simulink model "model"  (R2015a)
settings: Solver=ode3  StartTime=0.0  StopTime=30.0  RelTol=1e-3
undefined symbols (not defined in the file): MIO, National_Instruments, PCI
libraries: sldrtlib x3
settings Model: SimulationMode=external  ExtModeTrigDuration=1501  Creator=Alunos  LastModifiedBy=Alunos
settings HardwareCC: ProdIntDivRoundTo=Zero  ProdEndianess=LittleEndian  ProdHWDeviceType=Intel->x86/Pentium  TargetIntDivRoundTo=Zero  TargetEndianess=LittleEndian  TargetHWDeviceType=Intel->x86/Pentium
settings RTWCC: SystemTargetFile=rtwin.tlc  TemplateMakefile=rtwin.tmf  Description=Simulink Desktop Real-Time  RTWCompilerOptimization=on
settings CodeAppCC: MaxIdLength=95
settings RTWinTargetCC: TargetPreCompLibLocation=C:\Program Files\MATLAB\R2015a\toolbox\sldrt\lib\win32

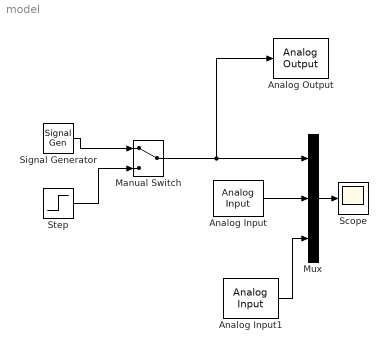
== system model ==
  Analog Input : sldrtlib/Analog Input  SampleTime=0.02  MaxMissedTicks=10  ShowMissedTicks=off  YieldWhenWaiting=off  DrvName=National_Instruments/PCI-MIO-16E-4  DrvAddress=4294967295  DrvOptions=[0 0 0 0 0 0]  Channels=1  RangeMode=1  VoltRange=1  DataType=1
      settings: AttributesFormatString=National Instruments\nPCI-MIO-16E-4 [auto]
  Analog Input1 : sldrtlib/Analog Input  SampleTime=0.02  MaxMissedTicks=10  ShowMissedTicks=off  YieldWhenWaiting=off  DrvName=National_Instruments/PCI-MIO-16E-4  DrvAddress=4294967295  DrvOptions=[0 0 0 0 0 0]  Channels=2  RangeMode=1  VoltRange=1  DataType=1
      settings: AttributesFormatString=National Instruments\nPCI-MIO-16E-4 [auto]
  Analog Output : sldrtlib/Analog Output  SampleTime=0.02  MaxMissedTicks=10  ShowMissedTicks=off  YieldWhenWaiting=off  DrvName=National_Instruments/PCI-MIO-16E-4  DrvAddress=4294967295  DrvOptions=[0 0 0 0 0 0]  Channels=1  RangeMode=1  VoltRange=1  InitialValue=0  FinalValue=0
      settings: AttributesFormatString=National Instruments\nPCI-MIO-16E-4 [auto]
  Manual Switch : ManualSwitch
  Mux : Mux  Inputs=3
  Scope : Scope
      settings: TickLabels=on  SaveName=input  SampleInput=on  SampleTime=0.02
  Signal Generator : SignalGenerator  WaveForm=square  Frequency=0.4
  Step : Step  SampleTime=0.02
  wires:
  Manual Switch/1 -> Mux/1, Analog Output/1
  Step/1 -> Manual Switch/2
  Analog Input1/1 -> Mux/3
  Analog Input/1 -> Mux/2
  Mux/1 -> Scope/1
  Signal Generator/1 -> Manual Switch/1
